simulink model "Desired_Shooting_Param_Calc"  (R2023b)
settings: Solver=FixedStepDiscrete  StartTime=0.0  StopTime=1  FixedStep=1  RelTol=1e-3
values from neighbouring files (symbols this model uses):
  isBlueAllianceTest = true    [Desired_Shooting_Param_Test.m]
  Robot_X_Test = Blue_Hub_X-2    [Desired_Shooting_Param_Test.m]
  Robot_Xv_Test = 0    [Desired_Shooting_Param_Test.m]
  Robot_Y_Test = Blue_Hub_Y-2    [Desired_Shooting_Param_Test.m]
  Robot_Yv_Test = 0    [Desired_Shooting_Param_Test.m]
settings Model: Creator=FIRSTMentor  LastModifiedBy=ander

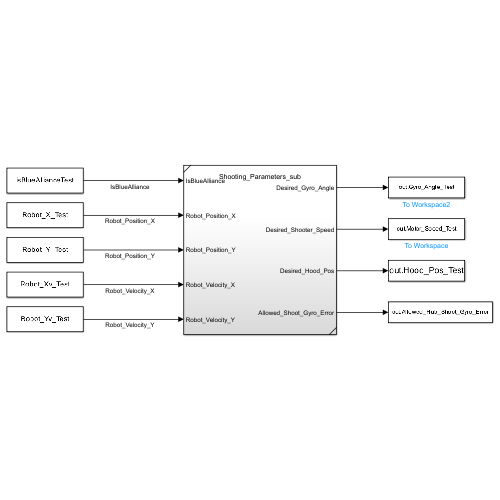
[thumbnail: Simulink's stored preview of the top-level diagram]
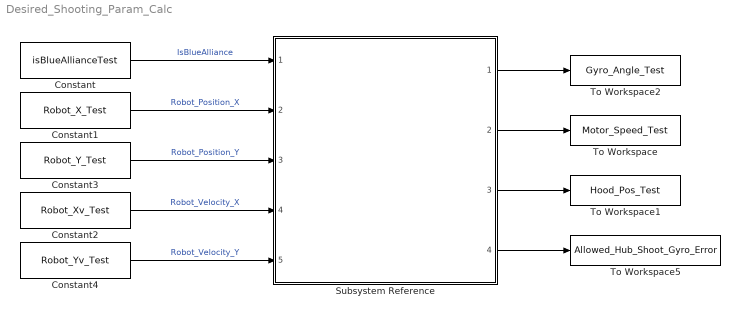
== system Desired_Shooting_Param_Calc ==
  Constant : Constant  Value=isBlueAllianceTest
  Constant1 : Constant  Value=Robot_X_Test
  Constant2 : Constant  Value=Robot_Xv_Test
  Constant3 : Constant  Value=Robot_Y_Test
  Constant4 : Constant  Value=Robot_Yv_Test
  Subsystem Reference : Subsystem  ReferencedSubsystem=Shooting_Parameters_sub
  To Workspace : ToWorkspace  VariableName=Motor_Speed_Test  SampleTime=-1
      settings: MaxDataPoints=1  Save2DSignal=2-D array (concatenate along first dimension)
  To Workspace1 : ToWorkspace  VariableName=Hood_Pos_Test  SampleTime=-1
      settings: MaxDataPoints=1
  To Workspace2 : ToWorkspace  VariableName=Gyro_Angle_Test  SampleTime=-1
      settings: MaxDataPoints=1
  To Workspace5 : ToWorkspace  VariableName=Allowed_Hub_Shoot_Gyro_Error  SampleTime=-1
      settings: MaxDataPoints=1
  wires:
  Constant/1 -> Subsystem Reference/1  "IsBlueAlliance"
  Constant1/1 -> Subsystem Reference/2  "Robot_Position_X"
  Constant2/1 -> Subsystem Reference/4  "Robot_Velocity_X"
  Constant3/1 -> Subsystem Reference/3  "Robot_Position_Y"
  Constant4/1 -> Subsystem Reference/5  "Robot_Velocity_Y"
  Subsystem Reference/1 -> To Workspace2/1
  Subsystem Reference/2 -> To Workspace/1
  Subsystem Reference/3 -> To Workspace1/1
  Subsystem Reference/4 -> To Workspace5/1
